simulink model "hovercraft_dynamic_control"  (R2024a)
settings: Solver=VariableStepAuto  StartTime=0.0  StopTime=30  RelTol=1e-3
values from neighbouring files (symbols this model uses):
  A = double(A)    [hovercraft_dynamic_lin.m]    (also in hovercraft_vel_dynamic_lin.m; mpc_vel.mat = [-0.1  0; 0  -0.05])
  B = double(B)    [hovercraft_dynamic_lin.m]    (also in hovercraft_vel_dynamic_lin.m; mpc_vel.mat = [1.11856823266  1.11856823266; 4  -4])
  C = [1 0 0 0 0 0; 0 0 1 0 0 0; 0 0 0 0 1 0]    [hovercraft_dynamic_lin.m]    (also in hovercraft_vel_dynamic_lin.m = [1 0; 0 1 ]; mpc_vel.mat = [1  0; 0  1])
  D = zeros(3,2)    [hovercraft_dynamic_lin.m]    (also in hovercraft_vel_dynamic_lin.m = zeros(2,2); mpc_vel.mat = [0  0; 0  0])
  Ts = 0.05    [hv_vel_opt.m]    (also in hv_vel_opt_lsqlin.m; mpc_vel.mat = 0.5)
  X0 = [0;0]    [hv_vel_opt.m]    (also in hv_vel_opt_lsqlin.m; mpc_vel.mat = [0 0])
libraries: mpclib x1
settings Model: Creator=ettor  LastModifiedBy=ettor

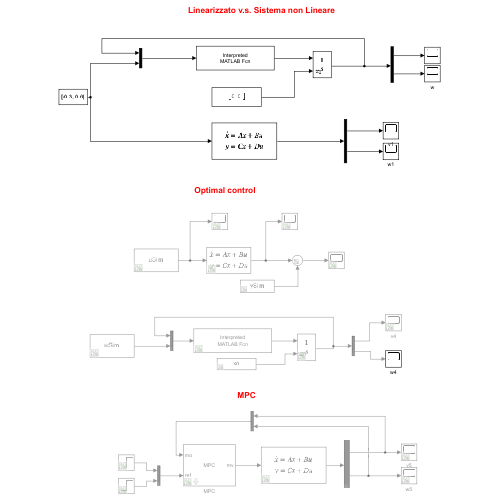
[thumbnail: Simulink's stored preview of the top-level diagram]
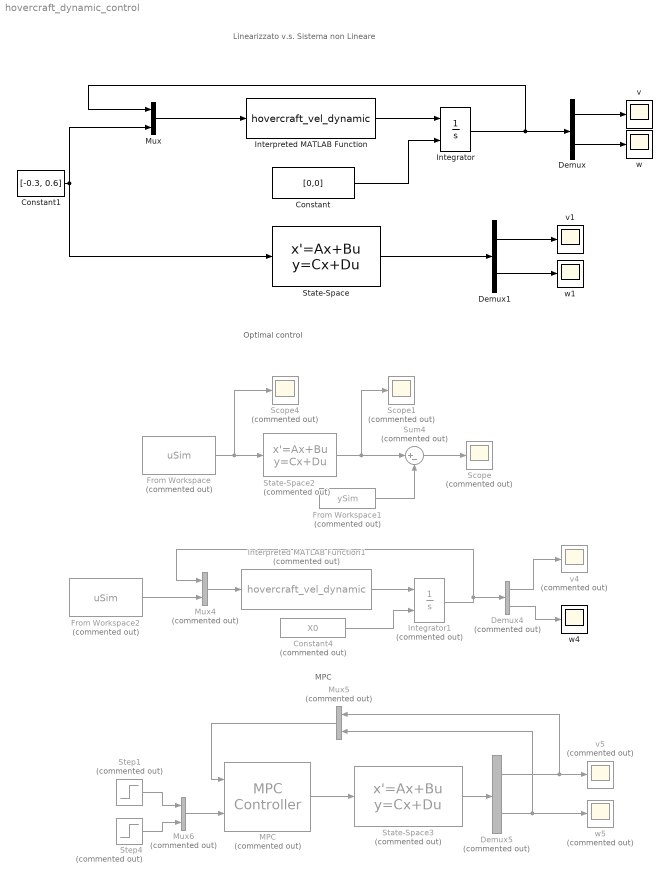
== system hovercraft_dynamic_control ==
  note: Linearizzato v.s. Sistema non Lineare
  note: Optimal control
  note: MPC
  Constant : Constant  Value=[0,0]
  Constant1 : Constant  Value=[-0.3, 0.6]
  Constant4 : Constant  Commented=on  Value=X0
  Demux : Demux  Outputs=2
  Demux1 : Demux  Outputs=2
  Demux4 : Demux  Commented=on  Outputs=2
  Demux5 : Demux  Commented=on  Outputs=2
  From Workspace : FromWorkspace  Commented=on  VariableName=uSim  SampleTime=Ts  OutputAfterFinalValue=Holding final value
  From Workspace1 : FromWorkspace  Commented=on  VariableName=ySim  SampleTime=Ts
  From Workspace2 : FromWorkspace  Commented=on  VariableName=uSim  SampleTime=Ts  OutputAfterFinalValue=Holding final value
  Integrator : Integrator  InitialConditionSource=external
  Integrator1 : Integrator  Commented=on  InitialConditionSource=external
  Interpreted MATLAB Function : MATLABFcn  MATLABFcn=hovercraft_vel_dynamic
  Interpreted MATLAB Function1 : MATLABFcn  Commented=on  MATLABFcn=hovercraft_vel_dynamic
  MPC : mpclib/MPC Controller  Commented=on  SCDEnableBlockLinearizationSpecification=on  mpcobj=mpc_vel  is_multiple=0  enable_value=0  return_u0=off  updateMPCinCallerWorkspace=on  md_inport=off  mv_inport=off  uref_inport=off  return_cost=off  return_mvseq=off  return_qpstatus=off  return_xseq=off  return_state=off  return_ovseq=off  state_inport=off  umin_inport=off  umax_inport=off  ymin_inport=off  ymax_inport=off  cc_inport=off  ywt_inport=off  uwt_inport=off  duwt_inport=off  rhoeps_inport=off  pm_inport=off  MaximumP=10  HorizonChoice=FixedHorizon  n_ts=0.05  n_p=80  n_mv=2  n_md=0  n_ud=0  n_mo=2  n_uo=0  BlockDataType=double  SampleTimeInherited=off  switch_inport=off
  Mux : Mux  Inputs=2
  Mux4 : Mux  Commented=on  Inputs=2
  Mux5 : Mux  Commented=on  Inputs=2
  Mux6 : Mux  Commented=on  Inputs=2
  Scope : Scope  Commented=on
  Scope1 : Scope  Commented=on
  Scope4 : Scope  Commented=on
  State-Space : StateSpace  A=A  B=B  C=C  D=D  InitialCondition=[0,0]
  State-Space2 : StateSpace  Commented=on  A=A  B=B  C=C  D=D  InitialCondition=X0
  State-Space3 : StateSpace  Commented=on  A=A  B=B  C=C  D=D  InitialCondition=[0,0]
  Step1 : Step  Commented=on  After=0.5  SampleTime=0.05
  Step4 : Step  Commented=on  Time=1.5  After=0.3  SampleTime=0.05
  Sum4 : Sum  Commented=on  Inputs=|+-
  v : Scope
  v1 : Scope
  v4 : Scope  Commented=on
  v5 : Scope  Commented=on
  w : Scope
  w1 : Scope
  w4 : Scope
  w5 : Scope  Commented=on
  wires:
  Constant/1 -> Integrator/2
  Mux/1 -> Interpreted MATLAB Function/1
  Constant1/1 -> State-Space/1, Mux/2
  Interpreted MATLAB Function/1 -> Integrator/1
  Integrator/1 -> Demux/1, Mux/1
  Demux/2 -> w/1
  Demux/1 -> v/1
  State-Space/1 -> Demux1/1
  Demux1/2 -> w1/1
  Demux1/1 -> v1/1
  From Workspace/1 -> Scope4/1, State-Space2/1
  From Workspace1/1 -> Sum4/2
  Sum4/1 -> Scope/1
  State-Space2/1 -> Sum4/1, Scope1/1
  Mux4/1 -> Interpreted MATLAB Function1/1
  Demux4/2 -> w4/1
  Demux4/1 -> v4/1
  Interpreted MATLAB Function1/1 -> Integrator1/1
  Integrator1/1 -> Mux4/1, Demux4/1
  Constant4/1 -> Integrator1/2
  From Workspace2/1 -> Mux4/2
  State-Space3/1 -> Demux5/1
  Demux5/2 -> Mux5/2, w5/1
  Demux5/1 -> Mux5/1, v5/1
  MPC/1 -> State-Space3/1
  Mux5/1 -> MPC/1
  Mux6/1 -> MPC/2
  Step4/1 -> Mux6/2
  Step1/1 -> Mux6/1
